simulink model "structure_impl_none"  (R2026b)
settings: Solver=VariableStepAuto
undefined symbols (not defined in the file or in its folder): P, Ts
libraries: fl_lib x1
settings Model: Creator=aomar  LastModifiedBy=aomar

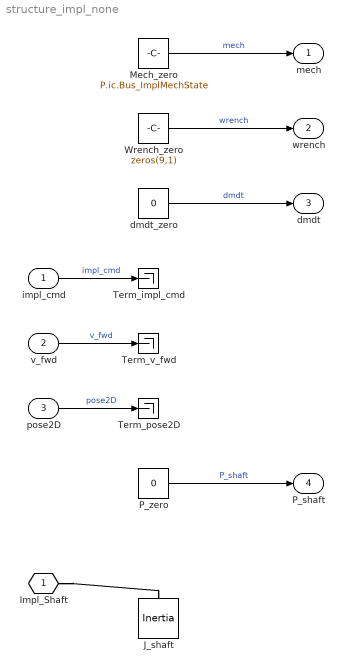
== system structure_impl_none ==
  impl_cmd : Inport  OutDataTypeStr=Bus: Bus_ImplementCmd  SampleTime=Ts.ctrl
  v_fwd : Inport  Port=2
  pose2D : Inport  Port=3
  J_shaft : fl_lib/Mechanical/Rotational Elements/Inertia  inertia=P.structure.impl.none.J kg*m^2  num_ports=foundation.enum.numPorts2.one  w_specify=off  w_priority=High  w=0 rad/s  w_nominal_specify=off  w_nominal_value=1  w_nominal_unit=rad/s  t_specify=off  t_priority=None  t=0 N*m  t_nominal_specify=off  t_nominal_value=1  t_nominal_unit=N*m
  Mech_zero : Constant  Value=P.ic.Bus_ImplMechState  VectorParams1D=off  OutDataTypeStr=Bus: Bus_ImplMechState
  P_zero : Constant  Value=0  VectorParams1D=off
  Term_impl_cmd : Terminator
  Term_pose2D : Terminator
  Term_v_fwd : Terminator
  Wrench_zero : Constant  Value=zeros(9,1)  VectorParams1D=off
  dmdt_zero : Constant  Value=0  VectorParams1D=off
  Impl_Shaft : PMIOPort  Side=Left  ConnectionType=Connection: foundation.mechanical.rotational.rotational
  mech : Outport  OutDataTypeStr=Bus: Bus_ImplMechState
  wrench : Outport  Port=2
  dmdt : Outport  Port=3
  P_shaft : Outport  Port=4
  wires:
  impl_cmd/1 -> Term_impl_cmd/1  "impl_cmd"
  v_fwd/1 -> Term_v_fwd/1  "v_fwd"
  pose2D/1 -> Term_pose2D/1  "pose2D"
  Mech_zero/1 -> mech/1  "mech"
  Wrench_zero/1 -> wrench/1  "wrench"
  dmdt_zero/1 -> dmdt/1  "dmdt"
  P_zero/1 -> P_shaft/1  "P_shaft"
  connections:
  Impl_Shaft/RConn1 -- J_shaft/LConn1
